simulink model "ecu_lamps"  (R2026a)
settings: Solver=FixedStepDiscrete  StopTime=10  FixedStep=0.001  SampleTimeConstraint=STIndependent
Description:
  | DM1 lamps: which faults light Protect. Source of truth for firmware/gen/ecu_lamps.
settings Model: Creator=jj1001000  LastModifiedBy=jj1001000
settings OptimizationCC: DefaultUnderspecifiedDataType=single
settings DebuggingCC: ParameterPrecisionLossMsg=none
settings HardwareCC: ProdLargestAtomicInteger=Long  ProdLargestAtomicFloat=Double  ProdHWDeviceType=ARM Compatible->ARM Cortex-M
settings RTWCC: SystemTargetFile=ert.tlc  GenCodeOnly=on  Description=Embedded Coder
settings ERTTargetCC: UtilityFuncGeneration=Shared location  IncludeMdlTerminateFcn=off  CodeInterfacePackaging=Reusable function  SupportNonFinite=off

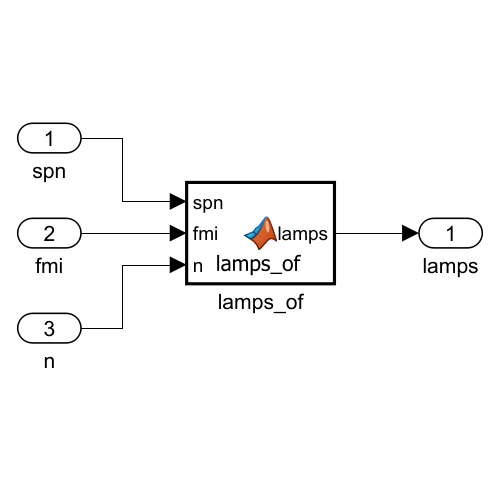
[thumbnail: Simulink's stored preview of the top-level diagram]
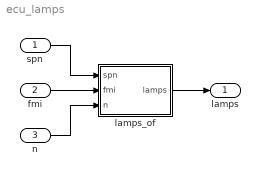
== system ecu_lamps ==
  spn : Inport  OutDataTypeStr=uint32  PortDimensions=16
  fmi : Inport  Port=2  OutDataTypeStr=uint8  PortDimensions=16
  n : Inport  Port=3  OutDataTypeStr=uint8
  lamps_of : MATLAB Function  TreatAsAtomicUnit=on
  lamps : Outport  OutDataTypeStr=uint8
  wires:
  spn/1 -> lamps_of/1(spn)
  n/1 -> lamps_of/3(n)
  fmi/1 -> lamps_of/2(fmi)
  lamps_of/1(lamps) -> lamps/1

== matlab function ecu_lamps/lamps_of ==
  data: spn input uint32; lamps output uint8; fmi input uint8; n input uint8
function lamps = lamps_of(spn, fmi, n)
%#codegen
lamps = uint8(0);
last = min(int32(n), int32(16));
for i = int32(1):last
    s = spn(i); f = fmi(i);
    if (s == uint32(190) && f == uint8(0)) || s == uint32(636) ...
            || (s == uint32(520192) && f == uint8(0)) || (s == uint32(110) && f == uint8(0))
        lamps = bitor(lamps, uint8(17));      % red + Protect: the DSE shuts down
    else
        lamps = bitor(lamps, uint8(4));      % amber
    end
end
